simulink model "M3_MeasuredLoop"  (R2026a)
settings: Solver=ode15s  StopTime=2  MaxStep=0.001
settings Model: Creator=siddh  LastModifiedBy=sjawahar

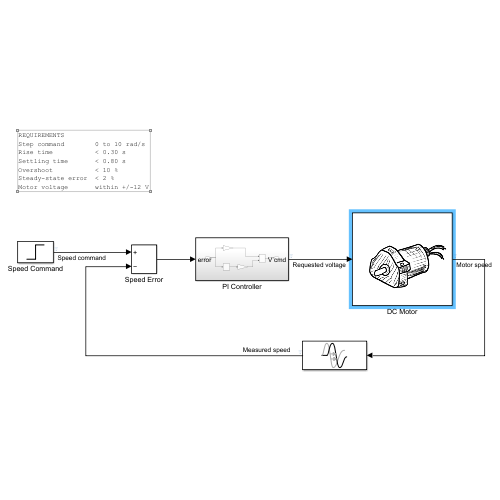
[thumbnail: Simulink's stored preview of the top-level diagram]
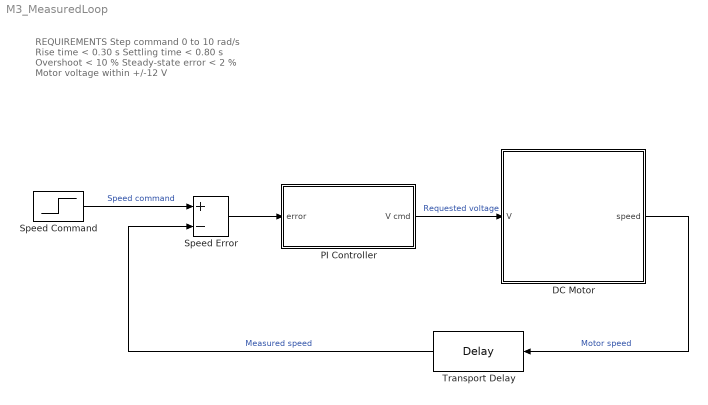
== system M3_MeasuredLoop ==
  note: REQUIREMENTS
      | Step command        0 to 10 rad/s
      | Rise time           < 0.30 s
      | Settling time       < 0.80 s
      | Overshoot           < 10 %
      | Steady-state error  < 2 %
      | Motor voltage       within +/-12 V
  DC Motor : Subsystem
      mask Display: image('DC motor.png')
  PI Controller : Subsystem
  Speed Command : Step  Time=0.1  FinalValue=10  SampleTime=0
  Speed Error : Sum  Inputs=+-
  Transport Delay : TransportDelay  DelayTime=0.06  PadeOrder=3
  wires:
  Speed Command/1 -> Speed Error/1  "Speed command"
  Speed Error/1 -> PI Controller/1(error)
  PI Controller/1(V cmd) -> DC Motor/1(V)  "Requested voltage"
  DC Motor/1(speed) -> Transport Delay/1  "Motor speed"
  Transport Delay/1 -> Speed Error/2  "Measured speed"

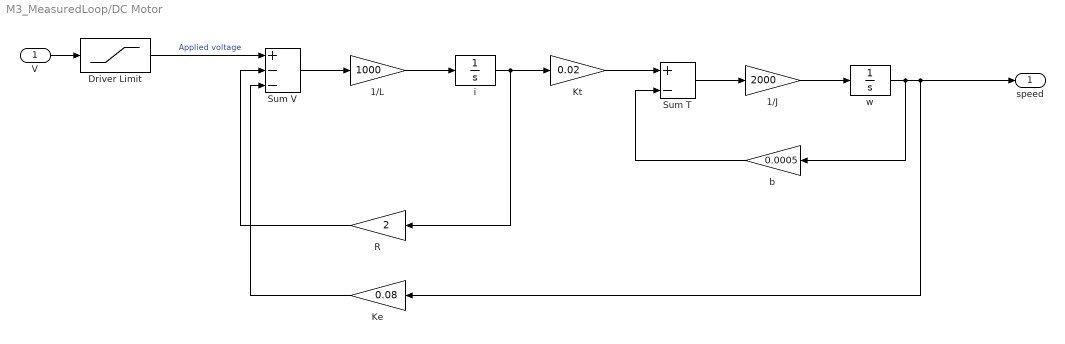
== system M3_MeasuredLoop/DC Motor ==
  V : Inport
  1/J : Gain  Gain=2000
  1/L : Gain  Gain=1000
  Driver Limit : Saturate  UpperLimit=12  LowerLimit=-12
  Ke : Gain  Gain=0.08
  Kt : Gain  Gain=0.02
  R : Gain  Gain=2
  Sum T : Sum  Inputs=+-
  Sum V : Sum  Inputs=+--
  b : Gain  Gain=0.0005
  i : Integrator
  w : Integrator
  speed : Outport
  wires:
  V/1 -> Driver Limit/1
  Driver Limit/1 -> Sum V/1  "Applied voltage"
  Sum V/1 -> 1/L/1
  1/L/1 -> i/1
  i/1 -> Kt/1, R/1
  Kt/1 -> Sum T/1
  Sum T/1 -> 1/J/1
  1/J/1 -> w/1
  w/1 -> speed/1, Ke/1, b/1
  b/1 -> Sum T/2
  R/1 -> Sum V/2
  Ke/1 -> Sum V/3

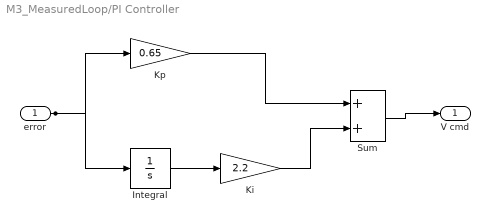
== system M3_MeasuredLoop/PI Controller ==
  error : Inport
  Integral : Integrator
  Ki : Gain  Gain=2.2
  Kp : Gain  Gain=0.65
  Sum : Sum
  V cmd : Outport
  wires:
  error/1 -> Kp/1, Integral/1
  Integral/1 -> Ki/1
  Kp/1 -> Sum/1
  Ki/1 -> Sum/2
  Sum/1 -> V cmd/1
